simulink model "AFC_FFNN_trainscg_15_15_15_15_15_Nor_July_15_RepCont"  (R2021a)
settings: Solver=ode15s  StartTime=0.0  StopTime=T  MaxStep=.01  RelTol=1e-3
InitFcn:
  | ensure_patch_sig_in();
undefined symbols (not defined in the file): AF_sensor_tol, fault_time, fuel_inj_tol, kappa_tol, MAF_sensor_tol, pump_tol, tau_ww_tol, x_gain, x_offset, y_gain, y_offset
libraries: neural x82
(part 2 of 4)

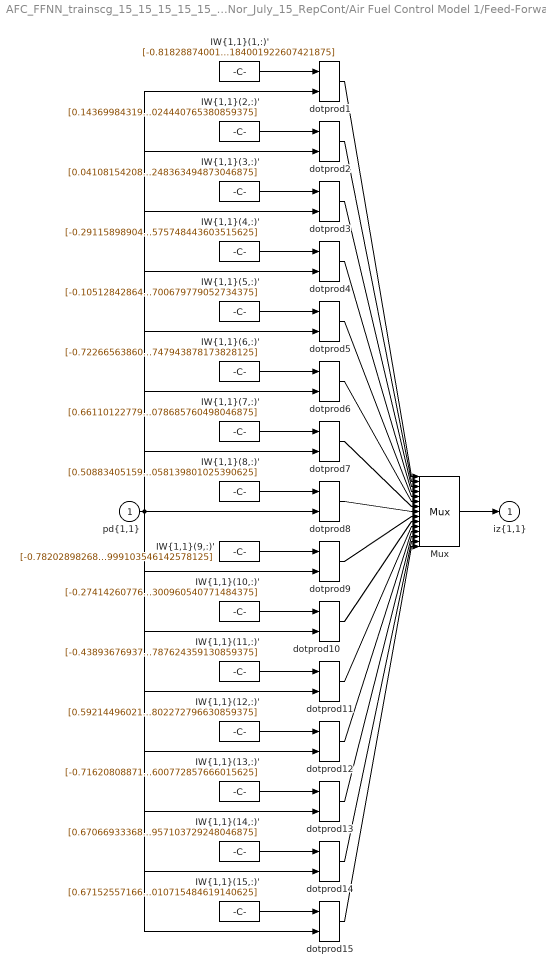
== system AFC_FFNN_trainscg_15_15_15_15_15_Nor_July_15_RepCont/Air Fuel Control Model 1/Feed-Forward Neural Network/Layer 1/IW{1,1} ==
  "pd{1,1}" : Inport  PortDimensions=4
      mask Display: e = 0.06;c1 = [120 230 180]/255;c2 = ([120 230 180]+0)/(256+128);c3 = ([120 230 180]+128)/(256+128);patch([0 1 1 0],[0 0 1 1],c1);patch([0 1 1 1-e 1-e 0+e],[0 0 1 1-e 0+e 0+e],c2);patch([0 0 1 1-e 0+e 0+e],[0 1 1 1-e 1-e 0+e],c3);plot([0 1 1 0 0],[0 0 1 1 0]);
  "IW{1,1}(1,:)'" : Constant  Value=[-0.8182887400167964120356600687955506145954132080078125;-0.49598144760943763120764060658984817564487457275390625;0.06041818616274809150556990289260284043848514556884765625;0.0133499737911447029226064131535167689435184001922607421875]
      mask Display: e = 0.06;c1 = [120 150 230]/255;c2 = ([120 150 230]+0)/383;c3 = ([120 150 230]+128)/383;patch([0 1 1 0],[0 0 1 1],c1);patch([0 1 1 1-e 1-e 0+e],[0 0 1 1-e 0+e 0+e],c2);patch([0 0 1 1-e 0+e 0+e],[0 1 1 1-e 1-e 0+e],c3);plot([0 1 1 0 0],[0 0 1 1 0]);disp('Weights');
  "IW{1,1}(10,:)'" : Constant  Value=[-0.274142607765400503350150529513484798371791839599609375;-0.353746335085151131227831911019166000187397003173828125;0.01179470110379924295551656854286193265579640865325927734375;0.099327920447423723171453957547782920300960540771484375]
      mask Display: e = 0.06;c1 = [120 150 230]/255;c2 = ([120 150 230]+0)/383;c3 = ([120 150 230]+128)/383;patch([0 1 1 0],[0 0 1 1],c1);patch([0 1 1 1-e 1-e 0+e],[0 0 1 1-e 0+e 0+e],c2);patch([0 0 1 1-e 0+e 0+e],[0 1 1 1-e 1-e 0+e],c3);plot([0 1 1 0 0],[0 0 1 1 0]);disp('Weights');
  "IW{1,1}(11,:)'" : Constant  Value=[-0.43893676937472270171980426312074996531009674072265625;0.1821822685096182448116763907819404266774654388427734375;0.69701670852280350754170967775280587375164031982421875;0.2445157951983446265042942968648276291787624359130859375]
      mask Display: e = 0.06;c1 = [120 150 230]/255;c2 = ([120 150 230]+0)/383;c3 = ([120 150 230]+128)/383;patch([0 1 1 0],[0 0 1 1],c1);patch([0 1 1 1-e 1-e 0+e],[0 0 1 1-e 0+e 0+e],c2);patch([0 0 1 1-e 0+e 0+e],[0 1 1 1-e 1-e 0+e],c3);plot([0 1 1 0 0],[0 0 1 1 0]);disp('Weights');
  "IW{1,1}(12,:)'" : Constant  Value=[0.59214496021067664077719427950796671211719512939453125;0.6211639297454680797017090299050323665142059326171875;0.45896429957388862330702750114141963422298431396484375;-0.71788574130490656610703581463894806802272796630859375]
      mask Display: e = 0.06;c1 = [120 150 230]/255;c2 = ([120 150 230]+0)/383;c3 = ([120 150 230]+128)/383;patch([0 1 1 0],[0 0 1 1],c1);patch([0 1 1 1-e 1-e 0+e],[0 0 1 1-e 0+e 0+e],c2);patch([0 0 1 1-e 0+e 0+e],[0 1 1 1-e 1-e 0+e],c3);plot([0 1 1 0 0],[0 0 1 1 0]);disp('Weights');
  "IW{1,1}(13,:)'" : Constant  Value=[-0.71620808871012420215862448458210565149784088134765625;0.4135587801428910470491473461152054369449615478515625;-0.289173209515923457235686555577558465301990509033203125;0.27039922822216144737694776267744600772857666015625]
      mask Display: e = 0.06;c1 = [120 150 230]/255;c2 = ([120 150 230]+0)/383;c3 = ([120 150 230]+128)/383;patch([0 1 1 0],[0 0 1 1],c1);patch([0 1 1 1-e 1-e 0+e],[0 0 1 1-e 0+e 0+e],c2);patch([0 0 1 1-e 0+e 0+e],[0 1 1 1-e 1-e 0+e],c3);plot([0 1 1 0 0],[0 0 1 1 0]);disp('Weights');
  "IW{1,1}(14,:)'" : Constant  Value=[0.67066933368885639499268336294335313141345977783203125;-0.453403126912178933149988324657897464931011199951171875;0.436183395002791851613466178605449385941028594970703125;0.4514754352094623168767384413513354957103729248046875]
      mask Display: e = 0.06;c1 = [120 150 230]/255;c2 = ([120 150 230]+0)/383;c3 = ([120 150 230]+128)/383;patch([0 1 1 0],[0 0 1 1],c1);patch([0 1 1 1-e 1-e 0+e],[0 0 1 1-e 0+e 0+e],c2);patch([0 0 1 1-e 0+e 0+e],[0 1 1 1-e 1-e 0+e],c3);plot([0 1 1 0 0],[0 0 1 1 0]);disp('Weights');
  "IW{1,1}(15,:)'" : Constant  Value=[0.6715255716655617046484394450089894235134124755859375;-0.887666042934819099485821425332687795162200927734375;-0.9589525699076890674632522859610617160797119140625;0.6290601453291844169513069573440589010715484619140625]
      mask Display: e = 0.06;c1 = [120 150 230]/255;c2 = ([120 150 230]+0)/383;c3 = ([120 150 230]+128)/383;patch([0 1 1 0],[0 0 1 1],c1);patch([0 1 1 1-e 1-e 0+e],[0 0 1 1-e 0+e 0+e],c2);patch([0 0 1 1-e 0+e 0+e],[0 1 1 1-e 1-e 0+e],c3);plot([0 1 1 0 0],[0 0 1 1 0]);disp('Weights');
  "IW{1,1}(2,:)'" : Constant  Value=[0.143699843190639720003076718057855032384395599365234375;-0.5405720325094571787616359870298765599727630615234375;-0.1096442863057018046735180405448772944509983062744140625;0.473688297171214356406920842346153222024440765380859375]
      mask Display: e = 0.06;c1 = [120 150 230]/255;c2 = ([120 150 230]+0)/383;c3 = ([120 150 230]+128)/383;patch([0 1 1 0],[0 0 1 1],c1);patch([0 1 1 1-e 1-e 0+e],[0 0 1 1-e 0+e 0+e],c2);patch([0 0 1 1-e 0+e 0+e],[0 1 1 1-e 1-e 0+e],c3);plot([0 1 1 0 0],[0 0 1 1 0]);disp('Weights');
  "IW{1,1}(3,:)'" : Constant  Value=[0.041081542089265621342519807512871921062469482421875;0.4871879533887997215657605920569039881229400634765625;-0.67363537454960553674254697398282587528228759765625;-0.2916475681070547221196420650812797248363494873046875]
      mask Display: e = 0.06;c1 = [120 150 230]/255;c2 = ([120 150 230]+0)/383;c3 = ([120 150 230]+128)/383;patch([0 1 1 0],[0 0 1 1],c1);patch([0 1 1 1-e 1-e 0+e],[0 0 1 1-e 0+e 0+e],c2);patch([0 0 1 1-e 0+e 0+e],[0 1 1 1-e 1-e 0+e],c3);plot([0 1 1 0 0],[0 0 1 1 0]);disp('Weights');
  "IW{1,1}(4,:)'" : Constant  Value=[-0.291158989040041060736285771781695075333118438720703125;0.85523357857572823714775722692138515412807464599609375;-0.343301083616170232826192432185052894055843353271484375;-0.164412991500933414190654957565129734575748443603515625]
      mask Display: e = 0.06;c1 = [120 150 230]/255;c2 = ([120 150 230]+0)/383;c3 = ([120 150 230]+128)/383;patch([0 1 1 0],[0 0 1 1],c1);patch([0 1 1 1-e 1-e 0+e],[0 0 1 1-e 0+e 0+e],c2);patch([0 0 1 1-e 0+e 0+e],[0 1 1 1-e 1-e 0+e],c3);plot([0 1 1 0 0],[0 0 1 1 0]);disp('Weights');
  "IW{1,1}(5,:)'" : Constant  Value=[-0.105128428648296246006310639131697826087474822998046875;0.365061060573851070554241005083895288407802581787109375;0.8346276011325670651785912923514842987060546875;0.09515404071335274716059160482473089359700679779052734375]
      mask Display: e = 0.06;c1 = [120 150 230]/255;c2 = ([120 150 230]+0)/383;c3 = ([120 150 230]+128)/383;patch([0 1 1 0],[0 0 1 1],c1);patch([0 1 1 1-e 1-e 0+e],[0 0 1 1-e 0+e 0+e],c2);patch([0 0 1 1-e 0+e 0+e],[0 1 1 1-e 1-e 0+e],c3);plot([0 1 1 0 0],[0 0 1 1 0]);disp('Weights');
  "IW{1,1}(6,:)'" : Constant  Value=[-0.722665638608478655413591695833019912242889404296875;0.985695769868679239067432718002237379550933837890625;-0.430803036254950644234895662521012127399444580078125;-0.8468350786113305606050971618969924747943878173828125]
      mask Display: e = 0.06;c1 = [120 150 230]/255;c2 = ([120 150 230]+0)/383;c3 = ([120 150 230]+128)/383;patch([0 1 1 0],[0 0 1 1],c1);patch([0 1 1 1-e 1-e 0+e],[0 0 1 1-e 0+e 0+e],c2);patch([0 0 1 1-e 0+e 0+e],[0 1 1 1-e 1-e 0+e],c3);plot([0 1 1 0 0],[0 0 1 1 0]);disp('Weights');
  "IW{1,1}(7,:)'" : Constant  Value=[0.66110122779032021167466837141546420753002166748046875;0.82898282548024060378821786798653192818164825439453125;0.72451838656569245156191527712508104741573333740234375;0.74217279844588712744979375202092342078685760498046875]
      mask Display: e = 0.06;c1 = [120 150 230]/255;c2 = ([120 150 230]+0)/383;c3 = ([120 150 230]+128)/383;patch([0 1 1 0],[0 0 1 1],c1);patch([0 1 1 1-e 1-e 0+e],[0 0 1 1-e 0+e 0+e],c2);patch([0 0 1 1-e 0+e 0+e],[0 1 1 1-e 1-e 0+e],c3);plot([0 1 1 0 0],[0 0 1 1 0]);disp('Weights');
  "IW{1,1}(8,:)'" : Constant  Value=[0.50883405159613970258902782006771303713321685791015625;0.594873705997945645407298798090778291225433349609375;-0.4681697843469925235382333994493819773197174072265625;0.492204681578230884841929082540445961058139801025390625]
      mask Display: e = 0.06;c1 = [120 150 230]/255;c2 = ([120 150 230]+0)/383;c3 = ([120 150 230]+128)/383;patch([0 1 1 0],[0 0 1 1],c1);patch([0 1 1 1-e 1-e 0+e],[0 0 1 1-e 0+e 0+e],c2);patch([0 0 1 1-e 0+e 0+e],[0 1 1 1-e 1-e 0+e],c3);plot([0 1 1 0 0],[0 0 1 1 0]);disp('Weights');
  "IW{1,1}(9,:)'" : Constant  Value=[-0.78202898268480403043412252372945658862590789794921875;0.85507523981980348981579709288780577480792999267578125;0.270272157299210558090152289878460578620433807373046875;-0.57478282284230808318881145169143564999103546142578125]
      mask Display: e = 0.06;c1 = [120 150 230]/255;c2 = ([120 150 230]+0)/383;c3 = ([120 150 230]+128)/383;patch([0 1 1 0],[0 0 1 1],c1);patch([0 1 1 1-e 1-e 0+e],[0 0 1 1-e 0+e 0+e],c2);patch([0 0 1 1-e 0+e 0+e],[0 1 1 1-e 1-e 0+e],c3);plot([0 1 1 0 0],[0 0 1 1 0]);disp('Weights');
  Mux : Mux  Inputs=15
      mask Display: e = 0.06;c1 = [120 150 230]/255;c2 = ([120 150 230]+0)/383;c3 = ([120 150 230]+128)/383;patch([0 1 1 0],[0 0 1 1],c1);patch([0 1 1 1-e 1-e 0+e],[0 0 1 1-e 0+e 0+e],c2);patch([0 0 1 1-e 0+e 0+e],[0 1 1 1-e 1-e 0+e],c3);plot([0 1 1 0 0],[0 0 1 1 0]);disp('Mux');
  dotprod{1..15} (15 alike) : neural/Weight Functions/dotprod
  "iz{1,1}" : Outport
      mask Display: e = 0.06;c1 = [120 230 180]/255;c2 = ([120 230 180]+0)/(256+128);c3 = ([120 230 180]+128)/(256+128);patch([0 1 1 0],[0 0 1 1],c1);patch([0 1 1 1-e 1-e 0+e],[0 0 1 1-e 0+e 0+e],c2);patch([0 0 1 1-e 0+e 0+e],[0 1 1 1-e 1-e 0+e],c3);plot([0 1 1 0 0],[0 0 1 1 0]);
  wires:
  Mux/1 -> "iz{1,1}"/1
  dotprod15/1 -> Mux/15
  "IW{1,1}(15,:)'"/1 -> dotprod15/1
  dotprod14/1 -> Mux/14
  "IW{1,1}(14,:)'"/1 -> dotprod14/1
  dotprod13/1 -> Mux/13
  "IW{1,1}(13,:)'"/1 -> dotprod13/1
  dotprod12/1 -> Mux/12
  "IW{1,1}(12,:)'"/1 -> dotprod12/1
  dotprod11/1 -> Mux/11
  "IW{1,1}(11,:)'"/1 -> dotprod11/1
  dotprod10/1 -> Mux/10
  "IW{1,1}(10,:)'"/1 -> dotprod10/1
  dotprod9/1 -> Mux/9
  "IW{1,1}(9,:)'"/1 -> dotprod9/1
  dotprod8/1 -> Mux/8
  "IW{1,1}(8,:)'"/1 -> dotprod8/1
  dotprod7/1 -> Mux/7
  "IW{1,1}(7,:)'"/1 -> dotprod7/1
  dotprod6/1 -> Mux/6
  "IW{1,1}(6,:)'"/1 -> dotprod6/1
  dotprod5/1 -> Mux/5
  "IW{1,1}(5,:)'"/1 -> dotprod5/1
  dotprod4/1 -> Mux/4
  "IW{1,1}(4,:)'"/1 -> dotprod4/1
  dotprod3/1 -> Mux/3
  "IW{1,1}(3,:)'"/1 -> dotprod3/1
  dotprod2/1 -> Mux/2
  "IW{1,1}(2,:)'"/1 -> dotprod2/1
  dotprod1/1 -> Mux/1
  "pd{1,1}"/1 -> dotprod15/2, dotprod14/2, dotprod13/2, dotprod12/2, dotprod11/2, dotprod10/2, dotprod9/2, dotprod8/2, dotprod7/2, dotprod6/2, dotprod5/2, dotprod4/2, dotprod3/2, dotprod2/2, dotprod1/2
  "IW{1,1}(1,:)'"/1 -> dotprod1/1

== system AFC_FFNN_trainscg_15_15_15_15_15_Nor_July_15_RepCont/Air Fuel Control Model 1/Feed-Forward Neural Network/Layer 2/Delays 1 ==
  "p{2}" : Inport  PortDimensions=15
      mask Display: e = 0.06;c1 = [120 230 180]/255;c2 = ([120 230 180]+0)/(256+128);c3 = ([120 230 180]+128)/(256+128);patch([0 1 1 0],[0 0 1 1],c1);patch([0 1 1 1-e 1-e 0+e],[0 0 1 1-e 0+e 0+e],c2);patch([0 0 1 1-e 0+e 0+e],[0 1 1 1-e 1-e 0+e],c3);plot([0 1 1 0 0],[0 0 1 1 0]);
  mux : Mux  Inputs=1
      mask Display: e = 0.06;c1 = [120 150 230]/255;c2 = ([120 150 230]+0)/383;c3 = ([120 150 230]+128)/383;patch([0 1 1 0],[0 0 1 1],c1);patch([0 1 1 1-e 1-e 0+e],[0 0 1 1-e 0+e 0+e],c2);patch([0 0 1 1-e 0+e 0+e],[0 1 1 1-e 1-e 0+e],c3);plot([0 1 1 0 0],[0 0 1 1 0]);disp('Mux')
  "pd{2,1}" : Outport
      mask Display: e = 0.06;c1 = [120 230 180]/255;c2 = ([120 230 180]+0)/(256+128);c3 = ([120 230 180]+128)/(256+128);patch([0 1 1 0],[0 0 1 1],c1);patch([0 1 1 1-e 1-e 0+e],[0 0 1 1-e 0+e 0+e],c2);patch([0 0 1 1-e 0+e 0+e],[0 1 1 1-e 1-e 0+e],c3);plot([0 1 1 0 0],[0 0 1 1 0]);
  wires:
  mux/1 -> "pd{2,1}"/1
  "p{2}"/1 -> mux/1

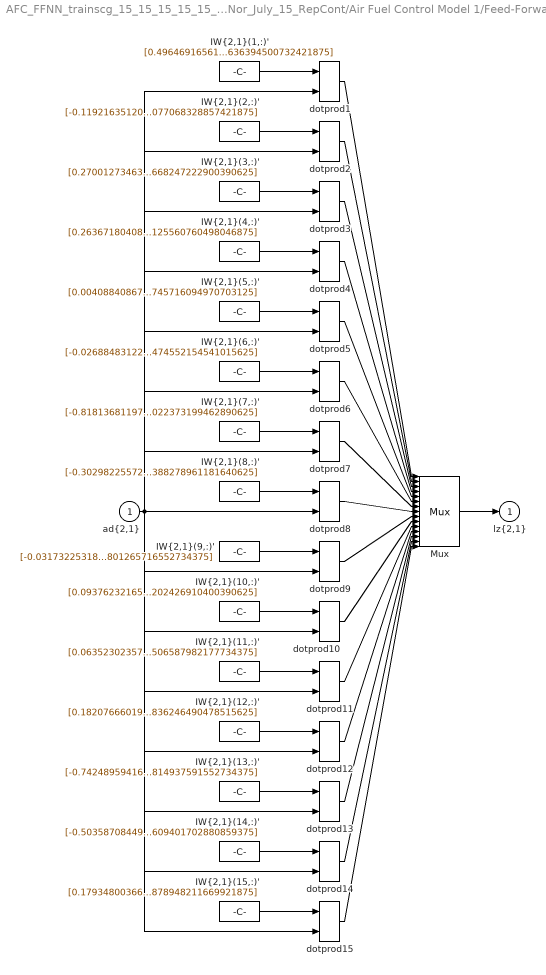
== system AFC_FFNN_trainscg_15_15_15_15_15_Nor_July_15_RepCont/Air Fuel Control Model 1/Feed-Forward Neural Network/Layer 2/LW{2,1} ==
  "ad{2,1}" : Inport  PortDimensions=15
      mask Display: e = 0.06;c1 = [120 230 180]/255;c2 = ([120 230 180]+0)/(256+128);c3 = ([120 230 180]+128)/(256+128);patch([0 1 1 0],[0 0 1 1],c1);patch([0 1 1 1-e 1-e 0+e],[0 0 1 1-e 0+e 0+e],c2);patch([0 0 1 1-e 0+e 0+e],[0 1 1 1-e 1-e 0+e],c3);plot([0 1 1 0 0],[0 0 1 1 0]);
  "IW{2,1}(1,:)'" : Constant  Value=[0.49646916561011245061507679565693251788616180419921875;0.77996133484927110401940808515064418315887451171875;-0.4843167782638080343105002611991949379444122314453125;0.91967297978227990906674449433921836316585540771484375;0.8707941521523403505256055723293684422969818115234375;0.5037557738819355979131842104834504425525665283203125;-0.7017295301971968601861817660392262041568756103515625;0.309274426520241119131782170370570383965969085693359375;0.90641457105355194290297049519722349941730499267578125;0.10882574325775402901417265866257366724312305450439453125;0.90673057127212108863290040972060523927211761474609375;-0.80524588547048792097626801478327251970767974853515625;0.104579561651616914641493849558173678815364837646484375;-0.386551898471740595919499128285679034888744354248046875;0.4908219201017736121883672240073792636394500732421875]
      mask Display: e = 0.06;c1 = [120 150 230]/255;c2 = ([120 150 230]+0)/383;c3 = ([120 150 230]+128)/383;patch([0 1 1 0],[0 0 1 1],c1);patch([0 1 1 1-e 1-e 0+e],[0 0 1 1-e 0+e 0+e],c2);patch([0 0 1 1-e 0+e 0+e],[0 1 1 1-e 1-e 0+e],c3);plot([0 1 1 0 0],[0 0 1 1 0]);disp('weights');
  "IW{2,1}(10,:)'" : Constant  Value=[0.0937623216569043460566490466590039432048797607421875;0.77106293047639129500936405747779645025730133056640625;0.4586134724193680067827472157659940421581268310546875;-0.7860483088632481685209540955838747322559356689453125;-0.52866293231569916333256742291268892586231231689453125;0.6383602490350686053943718434311449527740478515625;0.342034306689907363629998826581868343055248260498046875;0.212238388955804213598099750015535391867160797119140625;-0.976573937691504578850754114682786166667938232421875;0.64814439757751340920322036254219710826873779296875;-0.88015675771774992686147243148298002779483795166015625;-0.537524641968443628314844318083487451076507568359375;-0.552249744431198674732286235666833817958831787109375;-0.32473785236878993654130454160622321069240570068359375;-0.11032019079443211584390382995479740202426910400390625]
      mask Display: e = 0.06;c1 = [120 150 230]/255;c2 = ([120 150 230]+0)/383;c3 = ([120 150 230]+128)/383;patch([0 1 1 0],[0 0 1 1],c1);patch([0 1 1 1-e 1-e 0+e],[0 0 1 1-e 0+e 0+e],c2);patch([0 0 1 1-e 0+e 0+e],[0 1 1 1-e 1-e 0+e],c3);plot([0 1 1 0 0],[0 0 1 1 0]);disp('weights');
  "IW{2,1}(11,:)'" : Constant  Value=[0.06352302357512840114139862635056488215923309326171875;0.77580634612318088993987430512788705527782440185546875;0.4976683056216459899445681003271602094173431396484375;0.710615284497925880913271612371318042278289794921875;0.0284508200153920677577534803504022420383989810943603515625;-0.4262598504785959363516667508520185947418212890625;0.79535543465944924523824965945095755159854888916015625;-0.50420641521105835636262781918048858642578125;-0.78178862131788517952912798136821947991847991943359375;0.64520731580435242147331109663355164229869842529296875;0.8267663858165315016179874874069355428218841552734375;-0.480465110495678582314127424979233182966709136962890625;0.53645329785536877142959610864636488258838653564453125;0.09182180567506821600165523022951674647629261016845703125;-0.2422337966092920902294594043269171379506587982177734375]
      mask Display: e = 0.06;c1 = [120 150 230]/255;c2 = ([120 150 230]+0)/383;c3 = ([120 150 230]+128)/383;patch([0 1 1 0],[0 0 1 1],c1);patch([0 1 1 1-e 1-e 0+e],[0 0 1 1-e 0+e 0+e],c2);patch([0 0 1 1-e 0+e 0+e],[0 1 1 1-e 1-e 0+e],c3);plot([0 1 1 0 0],[0 0 1 1 0]);disp('weights');
  "IW{2,1}(12,:)'" : Constant  Value=[0.182076660191047789982832227906328625977039337158203125;0.0361498754295182800344576889983727596700191497802734375;0.943422814506380991161904603359289467334747314453125;-0.07051674807384201992821459725746535696089267730712890625;-0.91829558979760783632428911005263216793537139892578125;0.7502905528531134127234736297396011650562286376953125;0.496483911800009891646112691887537948787212371826171875;0.59923945203563711014993486969615332782268524169921875;-0.3292028577878360895425657872692681849002838134765625;-0.13105378107113896390956142568029463291168212890625;0.80434019538809276017587990281754173338413238525390625;0.249007566369504773629017790881334803998470306396484375;-0.89566786392105457448309380197315476834774017333984375;0.9758812474243507839588573915534652769565582275390625;-0.3177526207662977331125375712872482836246490478515625]
      mask Display: e = 0.06;c1 = [120 150 230]/255;c2 = ([120 150 230]+0)/383;c3 = ([120 150 230]+128)/383;patch([0 1 1 0],[0 0 1 1],c1);patch([0 1 1 1-e 1-e 0+e],[0 0 1 1-e 0+e 0+e],c2);patch([0 0 1 1-e 0+e 0+e],[0 1 1 1-e 1-e 0+e],c3);plot([0 1 1 0 0],[0 0 1 1 0]);disp('weights');
  "IW{2,1}(13,:)'" : Constant  Value=[-0.7424895941637081886455007406766526401042938232421875;-0.856648876074442622297056004754267632961273193359375;0.4489983138356112846167889074422419071197509765625;0.0342511534493581404348105934332124888896942138671875;-0.1478990255038865608838705156813375651836395263671875;-0.727415351703474044597896863706409931182861328125;-0.7367400157489829570778283596155233681201934814453125;0.0653226259463746128375305488589219748973846435546875;-0.089870329604618603980270563624799251556396484375;0.0129175888645709502355884978896938264369964599609375;0.8733140785372424108601308034849353134632110595703125;-0.2333190812499730260043406815384514629840850830078125;-0.72095782901882099480417309678159654140472412109375;-0.6008520238705161720105252243229188024997711181640625;-0.9615455944680115774048090315773151814937591552734375]
      mask Display: e = 0.06;c1 = [120 150 230]/255;c2 = ([120 150 230]+0)/383;c3 = ([120 150 230]+128)/383;patch([0 1 1 0],[0 0 1 1],c1);patch([0 1 1 1-e 1-e 0+e],[0 0 1 1-e 0+e 0+e],c2);patch([0 0 1 1-e 0+e 0+e],[0 1 1 1-e 1-e 0+e],c3);plot([0 1 1 0 0],[0 0 1 1 0]);disp('weights');
  "IW{2,1}(14,:)'" : Constant  Value=[-0.50358708449105638038645338383503258228302001953125;0.98956782330111947576511965962708927690982818603515625;-0.2361487675618059167703677303506992757320404052734375;0.007202825434977723484397671427359455265104770660400390625;-0.54195442663654513903992437917622737586498260498046875;0.95067385879104904233827255666255950927734375;-0.492871953524475603369836562706041149795055389404296875;-0.838459952423429744072791436337865889072418212890625;0.7937041538789466610381850841804407536983489990234375;0.59786126522488303169922119195689447224140167236328125;0.40169531108736389324320725791039876639842987060546875;-0.11999535239950331888536538826883770525455474853515625;0.3818939688303688573256522431620396673679351806640625;0.28629620337122674289531687463750131428241729736328125;0.306668631161549354313677895333967171609401702880859375]
      mask Display: e = 0.06;c1 = [120 150 230]/255;c2 = ([120 150 230]+0)/383;c3 = ([120 150 230]+128)/383;patch([0 1 1 0],[0 0 1 1],c1);patch([0 1 1 1-e 1-e 0+e],[0 0 1 1-e 0+e 0+e],c2);patch([0 0 1 1-e 0+e 0+e],[0 1 1 1-e 1-e 0+e],c3);plot([0 1 1 0 0],[0 0 1 1 0]);disp('weights');
  "IW{2,1}(15,:)'" : Constant  Value=[0.1793480036698109625348251938703469932079315185546875;-0.1774866557153116364276002059341408312320709228515625;0.0058018808544819666650482758996076881885528564453125;-0.43136233850821792401575294206850230693817138671875;0.6441880721956698696573084816918708384037017822265625;0.9393437732971190445852016637218184769153594970703125;-0.4988861248860751995692908167256973683834075927734375;0.1004589318309039303045437918626703321933746337890625;-0.874463826702308377747385748079977929592132568359375;0.301052562896285902382942367694340646266937255859375;-0.477452557381994768803679107804782688617706298828125;-0.759402127653759695391499917604960501194000244140625;-0.9407295984391181864481268348754383623600006103515625;-0.7407365473768721120251257161726243793964385986328125;0.8829622103937289079311767636681906878948211669921875]
      mask Display: e = 0.06;c1 = [120 150 230]/255;c2 = ([120 150 230]+0)/383;c3 = ([120 150 230]+128)/383;patch([0 1 1 0],[0 0 1 1],c1);patch([0 1 1 1-e 1-e 0+e],[0 0 1 1-e 0+e 0+e],c2);patch([0 0 1 1-e 0+e 0+e],[0 1 1 1-e 1-e 0+e],c3);plot([0 1 1 0 0],[0 0 1 1 0]);disp('weights');
  "IW{2,1}(2,:)'" : Constant  Value=[-0.11921635120059757839694469794267206452786922454833984375;-0.607546895104995154923699374194256961345672607421875;0.5900632710409168257825740511179901659488677978515625;-0.138270521887720487796968882321380078792572021484375;0.94863459152685891684342323060263879597187042236328125;0.108212254673193175591450199135579168796539306640625;0.6336456199801230315671318749082274734973907470703125;-0.852210835717297499058986431919038295745849609375;0.499621559800357439851126173380180262029170989990234375;0.324437729528092744235578948064357973635196685791015625;-0.450664172986721733860093763723853044211864471435546875;-0.53748757708461780691067133375327102839946746826171875;0.1466756409986354758867577174896723590791225433349609375;0.9207406241604727537009011939517222344875335693359375;0.6230024512652061474682341213338077068328857421875]
      mask Display: e = 0.06;c1 = [120 150 230]/255;c2 = ([120 150 230]+0)/383;c3 = ([120 150 230]+128)/383;patch([0 1 1 0],[0 0 1 1],c1);patch([0 1 1 1-e 1-e 0+e],[0 0 1 1-e 0+e 0+e],c2);patch([0 0 1 1-e 0+e 0+e],[0 1 1 1-e 1-e 0+e],c3);plot([0 1 1 0 0],[0 0 1 1 0]);disp('weights');
  "IW{2,1}(3,:)'" : Constant  Value=[0.2700127346397784844356237954343669116497039794921875;-0.9047528966046705090064961041207425296306610107421875;-0.430330309352361606300974017358385026454925537109375;-0.6030524532782468583036461495794355869293212890625;0.6380385707500888514687176211737096309661865234375;0.54795002035806472662216037861071527004241943359375;0.005250284302730445773477185866795480251312255859375;-0.1241388584709621767387943691574037075042724609375;-0.535917014359012622293221284053288400173187255859375;-0.7535723587361520259264580090530216693878173828125;-0.6954156221470046972399359219707548618316650390625;-0.1377055300142842053645608757506124675273895263671875;0.9674587418212110545567838926217518746852874755859375;-0.366043734123321140572215881547890603542327880859375;0.27252194091142545318007250898517668247222900390625]
      mask Display: e = 0.06;c1 = [120 150 230]/255;c2 = ([120 150 230]+0)/383;c3 = ([120 150 230]+128)/383;patch([0 1 1 0],[0 0 1 1],c1);patch([0 1 1 1-e 1-e 0+e],[0 0 1 1-e 0+e 0+e],c2);patch([0 0 1 1-e 0+e 0+e],[0 1 1 1-e 1-e 0+e],c3);plot([0 1 1 0 0],[0 0 1 1 0]);disp('weights');
  "IW{2,1}(4,:)'" : Constant  Value=[0.263671804087154904028267310422961600124835968017578125;-0.088848657628518290518826461266144178807735443115234375;0.319605914056265039135951155913062393665313720703125;0.43228381383499936418957076966762542724609375;-0.50480747820906402001384094546665437519550323486328125;0.5334080567160881525268223413149826228618621826171875;0.24319585957480349680537301537697203457355499267578125;0.0781634291431403394057042532949708402156829833984375;0.42457360577352798447492432387662120163440704345703125;0.419709979053071668975150032565579749643802642822265625;0.064052803186310125482805233332328498363494873046875;0.1443572233574179353166044847966986708343029022216796875;0.499054679010293267271691775022190995514392852783203125;-0.95638137624631947009135046755545772612094879150390625;0.73648140912501414145907574493321590125560760498046875]
      mask Display: e = 0.06;c1 = [120 150 230]/255;c2 = ([120 150 230]+0)/383;c3 = ([120 150 230]+128)/383;patch([0 1 1 0],[0 0 1 1],c1);patch([0 1 1 1-e 1-e 0+e],[0 0 1 1-e 0+e 0+e],c2);patch([0 0 1 1-e 0+e 0+e],[0 1 1 1-e 1-e 0+e],c3);plot([0 1 1 0 0],[0 0 1 1 0]);disp('weights');
  "IW{2,1}(5,:)'" : Constant  Value=[0.00408840867784126572870295746042756945826113224029541015625;0.09388048935012498208418918466122704558074474334716796875;-0.991924688688980982220755322487093508243560791015625;-0.8552316983080421319840525029576383531093597412109375;-0.1911860906079498878540334771969355642795562744140625;0.366618630720363825048480066470801830291748046875;0.7860653630786631484994586571701802313327789306640625;0.37038892020122304860052508956869132816791534423828125;-0.8905075787511116391925725110922940075397491455078125;-0.50182237106303106966009863754152320325374603271484375;0.7785018803667196340967393553000874817371368408203125;0.7206772319558594208643853562534786760807037353515625;-0.07958944169128155665671187080079107545316219329833984375;0.8513328940182223192323363036848604679107666015625;-0.9719425482959789253101234862697310745716094970703125]
      mask Display: e = 0.06;c1 = [120 150 230]/255;c2 = ([120 150 230]+0)/383;c3 = ([120 150 230]+128)/383;patch([0 1 1 0],[0 0 1 1],c1);patch([0 1 1 1-e 1-e 0+e],[0 0 1 1-e 0+e 0+e],c2);patch([0 0 1 1-e 0+e 0+e],[0 1 1 1-e 1-e 0+e],c3);plot([0 1 1 0 0],[0 0 1 1 0]);disp('weights');
  "IW{2,1}(6,:)'" : Constant  Value=[-0.0268848312263405588018461145338733331300318241119384765625;0.9246644738401335050781426616595126688480377197265625;-0.3050290799498984739557272405363619327545166015625;0.38414616541861434928506469077547080814838409423828125;0.034637294652763044033871864257889683358371257781982421875;0.625021902709288923460917430929839611053466796875;0.5043207504740092605999279840034432709217071533203125;0.1342838675116662938702205565277836285531520843505859375;-0.271313482373797321134389903818373568356037139892578125;0.4706688023118104080566581615130417048931121826171875;0.192185046668555903348618585368967615067958831787109375;0.903737226583765984599949661060236394405364990234375;-0.191130177012016011506290169563726522028446197509765625;-0.45184982043038257604194996019941754639148712158203125;-0.45605259254523444756301842062384821474552154541015625]
      mask Display: e = 0.06;c1 = [120 150 230]/255;c2 = ([120 150 230]+0)/383;c3 = ([120 150 230]+128)/383;patch([0 1 1 0],[0 0 1 1],c1);patch([0 1 1 1-e 1-e 0+e],[0 0 1 1-e 0+e 0+e],c2);patch([0 0 1 1-e 0+e 0+e],[0 1 1 1-e 1-e 0+e],c3);plot([0 1 1 0 0],[0 0 1 1 0]);disp('weights');
  "IW{2,1}(7,:)'" : Constant  Value=[-0.8181368119719962805902468971908092498779296875;-0.2417652257721003561385941793560050427913665771484375;0.77475446764487099216012211400084197521209716796875;-0.8479136503999418206234395256615243852138519287109375;-0.1962586542624291663372559924027882516384124755859375;-0.8289192649386392108823429225594736635684967041015625;-0.5728176091748220510879718858632259070873260498046875;-0.509054777740965302967879324569366872310638427734375;0.595048053803708398845628835260868072509765625;-0.0668896360863564520826685111387632787227630615234375;-0.723707884416889601908451368217356503009796142578125;-0.110236535200048280103146680630743503570556640625;-0.0815360751524158988701174166635610163211822509765625;-0.7837666978321446986655018918099813163280487060546875;0.676385977534560201007707291864790022373199462890625]
      mask Display: e = 0.06;c1 = [120 150 230]/255;c2 = ([120 150 230]+0)/383;c3 = ([120 150 230]+128)/383;patch([0 1 1 0],[0 0 1 1],c1);patch([0 1 1 1-e 1-e 0+e],[0 0 1 1-e 0+e 0+e],c2);patch([0 0 1 1-e 0+e 0+e],[0 1 1 1-e 1-e 0+e],c3);plot([0 1 1 0 0],[0 0 1 1 0]);disp('weights');
  "IW{2,1}(8,:)'" : Constant  Value=[-0.302982255725591453909828487667255103588104248046875;0.8981066832894628593209063183167017996311187744140625;0.7377501160157395876382224741973914206027984619140625;-0.51436050278973510785363032482564449310302734375;-0.974697580153902176647306987433694303035736083984375;0.7051429342498158892027504407451488077640533447265625;0.4605206164095310139572347907233051955699920654296875;-0.373094973925372386247545364312827587127685546875;0.162026455868859553532956851995550096035003662109375;0.0954318321609530784144226345233619213104248046875;-0.53521495323957424261607229709625244140625;-0.0899306950871696653138087640400044620037078857421875;-0.41688631732145697839087006286717951297760009765625;-0.75233462966951680783722622436471283435821533203125;-0.5567396324852271760619260021485388278961181640625]
      mask Display: e = 0.06;c1 = [120 150 230]/255;c2 = ([120 150 230]+0)/383;c3 = ([120 150 230]+128)/383;patch([0 1 1 0],[0 0 1 1],c1);patch([0 1 1 1-e 1-e 0+e],[0 0 1 1-e 0+e 0+e],c2);patch([0 0 1 1-e 0+e 0+e],[0 1 1 1-e 1-e 0+e],c3);plot([0 1 1 0 0],[0 0 1 1 0]);disp('weights');
  "IW{2,1}(9,:)'" : Constant  Value=[-0.03173225318246419845991113106720149517059326171875;-0.552686190513204333996100103831849992275238037109375;0.540447992482629313570896556484512984752655029296875;0.50729806833549417888207244686782360076904296875;-0.1229728520261097468591060533071868121623992919921875;0.612215314341371996675889022299088537693023681640625;-0.6820196650305467844788154252455569803714752197265625;0.7640746318530091674148252423037774860858917236328125;0.9475084056062905712991550899459980428218841552734375;0.406609182665139012868849022197537124156951904296875;-0.231903100212810020508413799689151346683502197265625;-0.83148171255660230372086516581475734710693359375;-0.5010392717716840582653503588517196476459503173828125;-0.443925165630052021015217178501188755035400390625;0.3313515085669587190153606570675037801265716552734375]
      mask Display: e = 0.06;c1 = [120 150 230]/255;c2 = ([120 150 230]+0)/383;c3 = ([120 150 230]+128)/383;patch([0 1 1 0],[0 0 1 1],c1);patch([0 1 1 1-e 1-e 0+e],[0 0 1 1-e 0+e 0+e],c2);patch([0 0 1 1-e 0+e 0+e],[0 1 1 1-e 1-e 0+e],c3);plot([0 1 1 0 0],[0 0 1 1 0]);disp('weights');
  Mux : Mux  Inputs=15
      mask Display: e = 0.06;c1 = [120 150 230]/255;c2 = ([120 150 230]+0)/383;c3 = ([120 150 230]+128)/383;patch([0 1 1 0],[0 0 1 1],c1);patch([0 1 1 1-e 1-e 0+e],[0 0 1 1-e 0+e 0+e],c2);patch([0 0 1 1-e 0+e 0+e],[0 1 1 1-e 1-e 0+e],c3);plot([0 1 1 0 0],[0 0 1 1 0]);disp('Mux');
  dotprod{1..15} (15 alike) : neural/Weight Functions/dotprod
  "lz{2,1}" : Outport
      mask Display: e = 0.06;c1 = [120 230 180]/255;c2 = ([120 230 180]+0)/(256+128);c3 = ([120 230 180]+128)/(256+128);patch([0 1 1 0],[0 0 1 1],c1);patch([0 1 1 1-e 1-e 0+e],[0 0 1 1-e 0+e 0+e],c2);patch([0 0 1 1-e 0+e 0+e],[0 1 1 1-e 1-e 0+e],c3);plot([0 1 1 0 0],[0 0 1 1 0]);
  wires:
  Mux/1 -> "lz{2,1}"/1
  dotprod15/1 -> Mux/15
  "IW{2,1}(15,:)'"/1 -> dotprod15/1
  dotprod14/1 -> Mux/14
  "IW{2,1}(14,:)'"/1 -> dotprod14/1
  dotprod13/1 -> Mux/13
  "IW{2,1}(13,:)'"/1 -> dotprod13/1
  dotprod12/1 -> Mux/12
  "IW{2,1}(12,:)'"/1 -> dotprod12/1
  dotprod11/1 -> Mux/11
  "IW{2,1}(11,:)'"/1 -> dotprod11/1
  dotprod10/1 -> Mux/10
  "IW{2,1}(10,:)'"/1 -> dotprod10/1
  dotprod9/1 -> Mux/9
  "IW{2,1}(9,:)'"/1 -> dotprod9/1
  dotprod8/1 -> Mux/8
  "IW{2,1}(8,:)'"/1 -> dotprod8/1
  dotprod7/1 -> Mux/7
  "IW{2,1}(7,:)'"/1 -> dotprod7/1
  dotprod6/1 -> Mux/6
  "IW{2,1}(6,:)'"/1 -> dotprod6/1
  dotprod5/1 -> Mux/5
  "IW{2,1}(5,:)'"/1 -> dotprod5/1
  dotprod4/1 -> Mux/4
  "IW{2,1}(4,:)'"/1 -> dotprod4/1
  dotprod3/1 -> Mux/3
  "IW{2,1}(3,:)'"/1 -> dotprod3/1
  dotprod2/1 -> Mux/2
  "IW{2,1}(2,:)'"/1 -> dotprod2/1
  dotprod1/1 -> Mux/1
  "ad{2,1}"/1 -> dotprod15/2, dotprod14/2, dotprod13/2, dotprod12/2, dotprod11/2, dotprod10/2, dotprod9/2, dotprod8/2, dotprod7/2, dotprod6/2, dotprod5/2, dotprod4/2, dotprod3/2, dotprod2/2, dotprod1/2
  "IW{2,1}(1,:)'"/1 -> dotprod1/1

== system AFC_FFNN_trainscg_15_15_15_15_15_Nor_July_15_RepCont/Air Fuel Control Model 1/Feed-Forward Neural Network/Layer 3/Delays 1 ==
  "p{3}" : Inport  PortDimensions=15
      mask Display: e = 0.06;c1 = [120 230 180]/255;c2 = ([120 230 180]+0)/(256+128);c3 = ([120 230 180]+128)/(256+128);patch([0 1 1 0],[0 0 1 1],c1);patch([0 1 1 1-e 1-e 0+e],[0 0 1 1-e 0+e 0+e],c2);patch([0 0 1 1-e 0+e 0+e],[0 1 1 1-e 1-e 0+e],c3);plot([0 1 1 0 0],[0 0 1 1 0]);
  mux : Mux  Inputs=1
      mask Display: e = 0.06;c1 = [120 150 230]/255;c2 = ([120 150 230]+0)/383;c3 = ([120 150 230]+128)/383;patch([0 1 1 0],[0 0 1 1],c1);patch([0 1 1 1-e 1-e 0+e],[0 0 1 1-e 0+e 0+e],c2);patch([0 0 1 1-e 0+e 0+e],[0 1 1 1-e 1-e 0+e],c3);plot([0 1 1 0 0],[0 0 1 1 0]);disp('Mux')
  "pd{3,2}" : Outport
      mask Display: e = 0.06;c1 = [120 230 180]/255;c2 = ([120 230 180]+0)/(256+128);c3 = ([120 230 180]+128)/(256+128);patch([0 1 1 0],[0 0 1 1],c1);patch([0 1 1 1-e 1-e 0+e],[0 0 1 1-e 0+e 0+e],c2);patch([0 0 1 1-e 0+e 0+e],[0 1 1 1-e 1-e 0+e],c3);plot([0 1 1 0 0],[0 0 1 1 0]);
  wires:
  mux/1 -> "pd{3,2}"/1
  "p{3}"/1 -> mux/1
